simulink model "wind_resource_standalone"  (R2023b)
settings: Solver=ode23t  StartTime=0.0  StopTime=1.0  MaxStep=1e-5  RelTol=1e-3
InitFcn:
  | root=fileparts(fileparts(fileparts(get_param(bdroot,'FileName')))); addpath(root); setup_v2_paths; define_resource_buses(true); define_v2_parameters(true); define_wind_test_fixture(true);
undefined symbols (not defined in the file): DiscIntNeverNeededParam, ee, GridTransformer, SM, Ts, V2
libraries: ee_lib x18, nesl_utility x17, fl_lib x5, eeSmAC1C x1
settings Model: Creator=fakebob2004  LastModifiedBy=fakebob2004
settings ModelReferenceCC: UpdateModelReferenceTargets=IfOutOfDate
settings RTWCC: GPUComputeCapability=5.0
settings ConfigComp: CovBoundaryAbsTol=1.0e-5
settings SimscapeCC: SimscapeNominalValues="[{\"value\":\"1\",\"unit\":\"A\"},{\"value\":\"1\",\"unit\":\"bar\"},{\"value\":\"1\",\"unit\":\"cm^2\"},{\"value\":\"1\",\"unit\":\"cm^3/s\"},{\"value\":\"1\",\"unit\":\"kJ/kg\"},{\"value\":\"1\",\"unit\":\"kW\"},{\"value\":\"1\",\"unit\":\"l\"},{\"value\":\"1\",\"unit\":\"N\"},{\"value\":\"1\",\"unit\":\"N*m\"},{\"value\":\"1\",\"unit\":\"V\"},{\"value\":\"0.001\",\"unit\":\"Wb\"}]"  SimscapeLogType=all  SimscapeLogDataHistory=10000

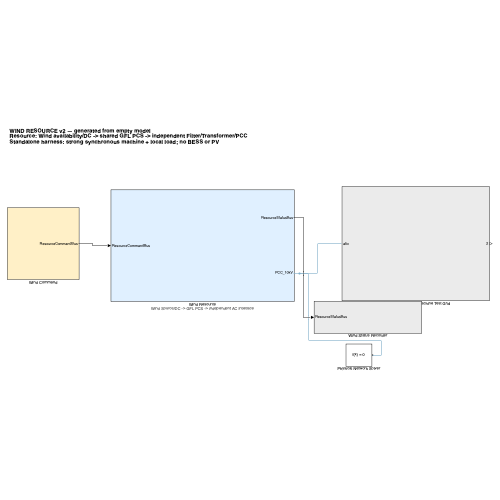
[thumbnail: Simulink's stored preview of the top-level diagram]
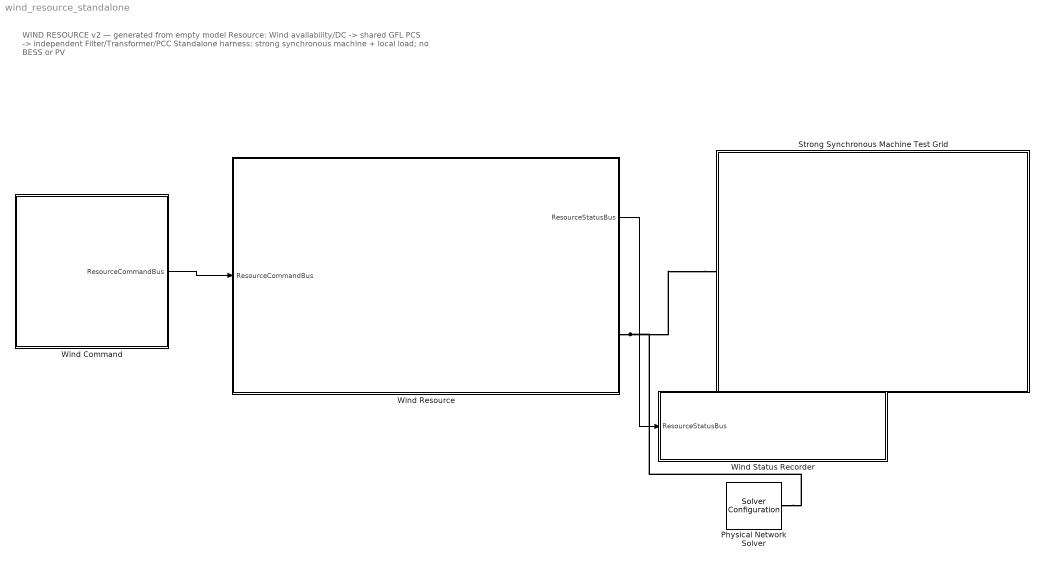
== system wind_resource_standalone ==
  note: WIND RESOURCE v2 — generated from empty model
      | Resource: Wind availability/DC -> shared GFL PCS -> independent Filter/Transformer/PCC
      | Standalone harness: strong synchronous machine + local load; no BESS or PV
  Physical Network Solver : nesl_utility/Solver Configuration  PhysicalDomain=network_engine_domain  SubClassName=solver  LeftPortType=input  RightPortType=generic  Tones=[]  Harmonics=[]  SimulateNoise=off  Profile=off  UseLocalSampling=off  EnableSwitchedLinearOptims=on  FrequencyDomain=off  UseCCode=off  RelTol=0.001  AbsTol=0.001  MinStep=1e-09  ToWorkspace=off  RevertToSquareIcSolve=off  NumHomotopyIterations=100  PhasorMode=off  PhasorModeNumHarmonics=1  ConsistencySolver=NEWTON_XTOL_AFTER_FTOL  CanonicalOrdering=CANONICAL  OptimizeIntermediates=OPTIMIZED  IndexReductionMethod=DerivativeReplacement  DoDC=off  ResidualTolerance=1e-09  ConsistencyTolSource=GLOBAL  ConsistencyAbsTol=0.001  ConsistencyRelTol=0.001  ConsistencyTolFactor=0.001  UseLocalSolver=off  LocalSolverChoice=NE_BACKWARD_EULER_ADVANCER  ResolveIndetEquations=on  FunctionEvalNumThread=1  LocalSolverSampleTime=0.001  DoFixedCost=off  MaxNonlinIter=3  MaxModeIter=2  ComputeImpulses=off  ImpulseIterations=2  LinearAlgebra=auto  LinearAlgebraNumThread=0  EquationFormulation=NE_TIME_EF  DelaysMemoryBudget=1024  AutomaticFiltering=on  FilteringTimeConstant=0.001  PartitionStorageMethod=AS_NEEDED  PartitionMemoryBudget=1024  PartitionMethod=ROBUST  MultibodyUseLocalSolver=off  MultibodyLocalSolverChoice=ODE1  MultibodyLocalSolverSampleTime=0.001
  Strong Synchronous Machine Test Grid : Subsystem  VariantControl=SynchronousMachine
  Wind Command : Subsystem
  Wind Resource : Subsystem
      settings: AttributesFormatString=Wind Source/DC -> GFL PCS -> independent AC Interface
  Wind Status Recorder : Subsystem
  wires:
  Wind Command/1(ResourceCommandBus) -> Wind Resource/1(ResourceCommandBus)
  Wind Resource/1(ResourceStatusBus) -> Wind Status Recorder/1(ResourceStatusBus)
  connections:
  Strong Synchronous Machine Test Grid/RConn1 -- Wind Resource/RConn1 -- Physical Network Solver/RConn1

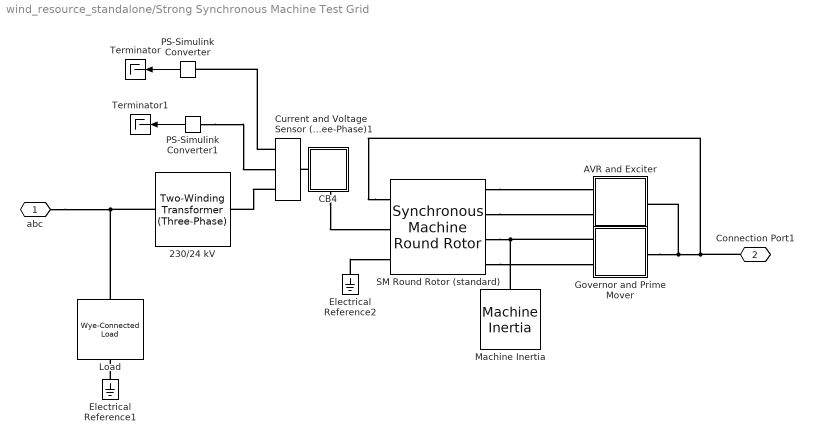
== system wind_resource_standalone/Strong Synchronous Machine Test Grid ==
  " Load" : ee_lib/Passive/RLC Assemblies/Wye-Connected Load  port_option=ee.enum.threePhasePort.composite  parameterization=ee.enum.rlc.parameterization.ratedpower  component_structure=ee.enum.rlc.structure.R  component_structure_PQ=ee.enum.rlc.structure.ParallelRL  R=1 Ohm  L=1e-3 H  C=1e-6 F  VRated=Grid.voltage V  FRated=Grid.frequency Hz  P=SM.P_load W  Qpos=SM.Q_load A*V  Qneg=-1e2 A*V  R_parasitic=0 Ohm  G_parasitic=0 1/Ohm  R_parasitic_PQ=0 Ohm  G_parasitic_PQ=0 1/Ohm  Vmag0=4.16e3 V  Vang0=0 deg  Freq0=60 Hz  IL_specify=off  IL_priority=High  IL=[0, 0, 0] A  IL_nominal_specify=off  IL_nominal_value=1  IL_nominal_unit=A  VC_specify=off  VC_priority=High  VC=[0, 0, 0] V  VC_nominal_specify=off  VC_nominal_value=1  VC_nominal_unit=V
  230/24 kV : ee_lib/Passive/Transformers/Two-Winding Transformer (Three-Phase)  SRated=SM.MVA V*A  FRated=Grid.frequency Hz  Winding1Connection=ee.enum.windingconnection.delta1  VRated1=Grid.voltage V  Winding2Connection=ee.enum.windingconnection.delta11  VRated2=SM.Voltage V  CoreType=ee.enum.coretype.fivelimb  pu_Rw1=GridTransformer.winding_resistance/2  pu_Rw2=GridTransformer.winding_resistance/2  leakage_reactance_option=ee.enum.transformer_leakage.include  pu_Xl1=GridTransformer.winding_lekage_reactance/2  pu_Xl2=GridTransformer.winding_lekage_reactance/2  magnetizing_resistance_option=ee.enum.transformer_magnetizingResistance.exclude  pu_Rm=500  magnetizing_reactance_option=ee.enum.transformer_magnetizingReactance.include  saturation_option=ee.enum.transformer_saturation.exclude  pu_Xm=500  current_data=[0, .002, 1, 2]  magnetic_flux_data=[0, 1.2, 1.5, 1.51]  pu_X0=0.0586/2  i1_specify=off  i1_priority=None  i1=[ 0 0 0 ] A  i1_nominal_specify=off  i1_nominal_value=1  i1_nominal_unit=A  i2_specify=off  i2_priority=None  i2=[ 0 0 0 ] A  i2_nominal_specify=off  i2_nominal_value=1  i2_nominal_unit=A  phi_specify=off  phi_priority=None  phi=[ 0 0 0 ]  phi_nominal_specify=off  phi_nominal_value=1  phi_nominal_unit=1
  AVR and Exciter : Subsystem
  CB4 : Subsystem
      settings: PortSchema="{\"entries\":[{\"content\":{\"sides\":[{\"content\":{\"connectorIds\":[\"LConn1\"]},\"type\":\"ConnectorPlacement.EquallySpacedRectSide\",\"uuid\":\"24022911-97b6-486c-a625-f0780a134feb\"},{\"content\":{\"connectorIds\":[],\"side\":\"RIGHT\"},\"type\":\"ConnectorPlacement.EquallySpacedRectSide\",\"uuid\":\"1242aa8b-343b-4af2-8b96-dfa58505a53d\"},{\"content\":{\"connectorIds\":[],\"side\":\"TOP\"},\"type\":\"ConnectorPlacement.EquallySpacedRectSide\",\"uuid\":\"e73be2e9-5300-480f-914f-665ff518f6ad\"},{\"content\":{\"connectorIds\":[\"RConn1\"],\"side\":\"BOTTOM\"},\"type\":\"ConnectorPlacement.EquallySpacedRectSide\",\"uuid\":\"6525202c-c4e7-4c96-9421-427b801d0594\"}]},\"type\":\"ConnectorPlacement.EquallySpacedConnector\",\"uuid\":\"b455682c-e951-4ef6-bff8-cd3f50b315f1\"}],\"packageUris\":[\"http://schema.mathworks.com/mf0/Connector/R2020b\"],\"version\":\"1.0\"}"
      mask Display: image('$imagefile'); % Use "Edit Image" on toolstrip to change.
  Current and Voltage Sensor (Three-Phase)1 : ee_lib/Sensors & Transducers/Current and Voltage Sensor (Three-Phase)  port_option=ee.enum.threePhasePort.composite  vMeasurementType=ee.enum.vmeasurement.ll  outputUnit=ee.enum.unit.pu  SRated=100e6 A*V  VRated=4.16e3 V  I_specify=off  I_priority=None  I=[0, 0, 0] A  I_nominal_specify=off  I_nominal_value=1  I_nominal_unit=A  V_specify=off  V_priority=None  V=[0, 0, 0] V  V_nominal_specify=off  V_nominal_value=1  V_nominal_unit=V
  Electrical Reference1 : fl_lib/Electrical/Electrical Elements/Electrical Reference
  Electrical Reference2 : fl_lib/Electrical/Electrical Elements/Electrical Reference
  "Governor and Prime Mover " : Subsystem  mask(Governor and Prime Mover){pu_speed_reference=SM.speed_reference, droop_percentage=SM.droop_p, pu_load_reference_setpoint=SM.load_reference_set_point, T_G=SM.governor_time_constant, T_CH=SM.time_constsnt_steamchest, base_torque=SM.Base_Torque_SM, pu_torque0=SM.initial_torque}
      mask prompts: pu_speed_reference "Speed reference, (pu)"; droop_percentage "Percentage droop, (%)"; pu_load_reference_setpoint "Load reference setpoint, (pu)"; T_G "Time constant of governor, (s)"; T_CH "Time constant of main inlet volumes and steam chest, (s)"; base_torque "Base torque, (N*m)"; pu_torque0 "Initial torque, (pu)"
      mask help:
      | Implements a synchronous machine governor and prime mover. The prime mover is a non-reheat steam turbine.
      |
      | The input to the block is a per-unit synchronous machine measurement vector.
      |
      | R and C are mechanical rotational ports.
  Machine Inertia : ee_lib/Electromechanical/Mechanical/Machine Inertia  SRated=SM.MVA V*A  FRated=Grid.frequency Hz  nPolePairs=SM.polepairs  inertia_option=2  J=27548 kg*m^2  H=SM.inertia s  damper_option=2  D=39.0509 N*m/(rad/s)  pu_D=SM.damping  initialization_option=2  fMechanical0=60 Hz  fElectrical0=Grid.frequency Hz
  PS-Simulink Converter : nesl_utility/PS-Simulink Converter  PhysicalDomain=network_engine_domain  SubClassName=ps_output  LeftPortType=input  RightPortType=output  PseudoPeriodic=off  Frequencies=[]  VectorFormat=inherit  Unit=inherit  AffineConversion=off
  PS-Simulink Converter1 : nesl_utility/PS-Simulink Converter  PhysicalDomain=network_engine_domain  SubClassName=ps_output  LeftPortType=input  RightPortType=output  PseudoPeriodic=off  Frequencies=[]  VectorFormat=inherit  Unit=inherit  AffineConversion=off
  SM Round Rotor (standard) : ee_lib/Electromechanical/Synchronous/Synchronous Machine Round Rotor  port_option=ee.enum.threePhasePort.composite  SRated=SM.MVA V*A  VRated=SM.Voltage V  FRated=Grid.frequency Hz  nPolePairs=SM.polepairs  param_option=ee.enum.sm.parameterization.standard  fieldCircuitParameterization_option=2  baseEfd=92.95 V  baseIfd=SM.field_current A  zero_sequence=ee.enum.park.zerosequence.include  axes_param=ee.enum.rotorangle.qaxis  Ladu=1.66  Laqu=1.61  L0=0.15  Ll=0.15  Ra=SM.stator_resistance  Lfd=0.165  Rfd=0.0006  L1d=0.1713  R1d=0.0284  L1q=0.7252  R1q=0.00619  L2q=0.125  R2q=0.02368  Xl=SM.lekage_reactance  Xd=SM.xd  Xq=SM.xq  X0=0.15  Xdd=SM.xd_  Xqd=SM.xq_  Xddd=SM.xd_dash  Xqdd=SM.xq_dash  d_option=1  Td0d=SM.Tdo_ s  Tdd=1.3260 s  Td0dd=SM.Tdo_dash s  Tddd=0.0230 s  q_option=1  Tq0d=SM.Tqo_ s  Tqd=0.3693 s  Tq0dd=SM.Tqo_dash s  Tqdd=0.0269 s  saturation_option=0  saturation_ifd=[0.00, 0.48, 0.76, 1.38, 1.79]  saturation_Vag=[0.00, 0.80, 1.08, 1.31, 1.40]  initialization_option=2  source_type=ee.enum.sm.load_flow_source_type.Swing  Vmag0=SM.Voltage V  Vang0=0 deg  Pt0=SM.initial_Pe V*A  Qt0=SM.initial_Qe V*A  minimum_pu=0.95  phase_search_range=[-inf, inf] deg  gmin=1e-6 S  connection_option=int32(ee.enum.Connection.wye)  num_q_dampers=2  rotor_offset=-pi / 2 rad  pu_psid_specify=on  pu_psid_priority=High  pu_psid=0  pu_psid_nominal_specify=off  pu_psid_nominal_value=1  pu_psid_nominal_unit=1  pu_psiq_specify=on  pu_psiq_priority=High  pu_psiq=0  pu_psiq_nominal_specify=off  pu_psiq_nominal_value=1  pu_psiq_nominal_unit=1  pu_psifd_specify=on  pu_psifd_priority=High  pu_psifd=0  pu_psifd_nominal_specify=off  pu_psifd_nominal_value=1  pu_psifd_nominal_unit=1  pu_psi1d_specify=on  pu_psi1d_priority=High  pu_psi1d=0  pu_psi1d_nominal_specify=off  pu_psi1d_nominal_value=1  pu_psi1d_nominal_unit=1  pu_psi1q_specify=on  pu_psi1q_priority=High  pu_psi1q=0  pu_psi1q_nominal_specify=off  pu_psi1q_nominal_value=1  pu_psi1q_nominal_unit=1  pu_psi2q_specify=on  pu_psi2q_priority=High  pu_psi2q=0  pu_psi2q_nominal_specify=off  pu_psi2q_nominal_value=1  pu_psi2q_nominal_unit=1  angular_position_diff_specify=on  angular_position_diff_priority=High  angular_position_diff=0 deg  angular_position_diff_nominal_specify=off  angular_position_diff_nominal_value=1  angular_position_diff_nominal_unit=deg  Tmeas=298.15 K  alpha=3.93e-3 1/K  stator_thermal_mass=100 J/K  rotor_thermal_mass=200 J/K  temperatureA_specify=off  temperatureA_priority=High  temperatureA=25 degC  temperatureA_nominal_specify=off  temperatureA_nominal_value=1  temperatureA_nominal_unit=degC  temperatureB_specify=off  temperatureB_priority=High  temperatureB=25 degC  temperatureB_nominal_specify=off  temperatureB_nominal_value=1  temperatureB_nominal_unit=degC  temperatureC_specify=off  temperatureC_priority=High  temperatureC=25 degC  temperatureC_nominal_specify=off  temperatureC_nominal_value=1  temperatureC_nominal_unit=degC  temperatureR_specify=off  temperatureR_priority=High  temperatureR=25 degC  temperatureR_nominal_specify=off  temperatureR_nominal_value=1  temperatureR_nominal_unit=degC
  Terminator : Terminator
  Terminator1 : Terminator
  abc : PMIOPort  Side=Right
  Connection Port1 : PMIOPort  Port=2  Side=Left
  wires:
  PS-Simulink Converter1/1 -> Terminator1/1
  PS-Simulink Converter/1 -> Terminator/1
  connections:
  Electrical Reference2/LConn1 -- SM Round Rotor (standard)/RConn3
  CB4/RConn1 -- SM Round Rotor (standard)/RConn2
  PS-Simulink Converter1/LConn1 -- Current and Voltage Sensor (Three-Phase)1/RConn2
  Current and Voltage Sensor (Three-Phase)1/RConn3 -- 230/24 kV/RConn1
  SM Round Rotor (standard)/LConn2 -- AVR and Exciter/RConn2
  Electrical Reference1/LConn1 -- " Load"/RConn1
  CB4/LConn1 -- Current and Voltage Sensor (Three-Phase)1/LConn1
  SM Round Rotor (standard)/LConn1 -- AVR and Exciter/RConn1
  Current and Voltage Sensor (Three-Phase)1/RConn1 -- PS-Simulink Converter/LConn1
  SM Round Rotor (standard)/LConn4 -- "Governor and Prime Mover "/RConn2
  "Governor and Prime Mover "/RConn1 -- Machine Inertia/LConn1 -- SM Round Rotor (standard)/LConn3
  SM Round Rotor (standard)/RConn1 -- Connection Port1/RConn1 -- AVR and Exciter/LConn1 -- "Governor and Prime Mover "/LConn1
  230/24 kV/LConn1 -- abc/RConn1 -- " Load"/LConn1

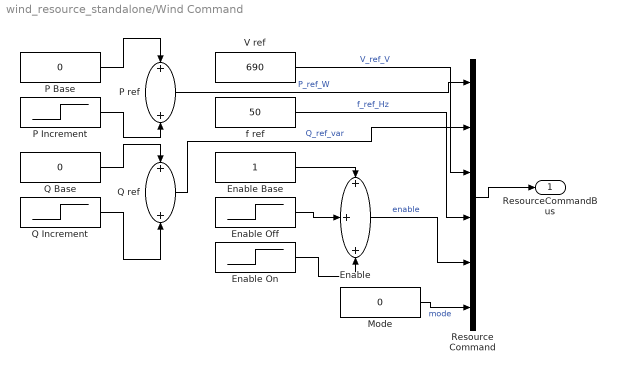
== system wind_resource_standalone/Wind Command ==
  Enable : Sum  Inputs=+++
  Enable Base : Constant
  Enable Off : Step  Time=10  After=-1  SampleTime=0
  Enable On : Step  Time=11  SampleTime=0
  Mode : Constant  Value=0
  P Base : Constant  Value=0
  P Increment : Step  Time=.30  After=2e6  SampleTime=0
  P ref : Sum
  Q Base : Constant  Value=0
  Q Increment : Step  Time=.30  After=0  SampleTime=0
  Q ref : Sum
  Resource Command : BusCreator  Inputs=6  OutDataTypeStr=Bus: ResourceCommandBus
  V ref : Constant  Value=690
  f ref : Constant  Value=50
  ResourceCommandBus : Outport  OutDataTypeStr=Bus: ResourceCommandBus
  wires:
  P Base/1 -> P ref/1
  P Increment/1 -> P ref/2
  Q Base/1 -> Q ref/1
  Q Increment/1 -> Q ref/2
  Enable Base/1 -> Enable/1
  Enable Off/1 -> Enable/2
  Enable On/1 -> Enable/3
  P ref/1 -> Resource Command/1  "P_ref_W"
  Q ref/1 -> Resource Command/2  "Q_ref_var"
  V ref/1 -> Resource Command/3  "V_ref_V"
  f ref/1 -> Resource Command/4  "f_ref_Hz"
  Enable/1 -> Resource Command/5  "enable"
  Mode/1 -> Resource Command/6  "mode"
  Resource Command/1 -> ResourceCommandBus/1

== system wind_resource_standalone/Wind Resource ==
  ResourceCommandBus : Inport  OutDataTypeStr=Bus: ResourceCommandBus
  01 Wind Source and DC Side : Subsystem
      settings: AttributesFormatString=replaceable by turbine + PMSG + MSC + physical DC link
  02 PCS : Subsystem
      settings: AttributesFormatString=local PLL | P/Q-to-dq | circle limit | average PCS
  03 AC Interface : Subsystem
      settings: AttributesFormatString=independent filter + 0.69/10 kV transformer + PCC sensing
  Status Interface : Subsystem
      settings: AttributesFormatString=typed local buses -> ResourceStatusBus
  PCC_10kV : PMIOPort  Side=Right  ConnectionType=Connection: foundation.electrical.three_phase
  ResourceStatusBus : Outport  OutDataTypeStr=Bus: ResourceStatusBus
  wires:
  ResourceCommandBus/1 -> 01 Wind Source and DC Side/1(ResourceCommandBus)
  01 Wind Source and DC Side/1(PCSCommandBus) -> 02 PCS/1(CommandBus)
  03 AC Interface/1(PCCMeasurementBus) -> 02 PCS/2(PCCMeasurementBus), Status Interface/3(PCC)
  01 Wind Source and DC Side/2(SourceStatusBus) -> Status Interface/1(Source)
  02 PCS/1(PCSStatusBus) -> Status Interface/2(PCS)
  Status Interface/1(ResourceStatusBus) -> ResourceStatusBus/1
  connections:
  02 PCS/RConn1 -- 03 AC Interface/LConn1
  03 AC Interface/RConn1 -- PCC_10kV/RConn1

== system wind_resource_standalone/Wind Status Recorder ==
  ResourceStatusBus : Inport  OutDataTypeStr=Bus: ResourceStatusBus
  Regression Vector : Mux  Inputs=12
  Status Selector : BusSelector  OutputSignals=P_W,Q_var,Vpcc_V,frequency_Hz,available_power_W,power_headroom_W,current_limit_factor,energy_state_pu,Vdc_V,control_mode,healthy
  Time : Clock
  Wind v2 Result : ToWorkspace  VariableName=wind_v2_result  SampleTime=-1
  wires:
  Time/1 -> Regression Vector/1
  Status Selector/1 -> Regression Vector/2  "<P_W>"
  Status Selector/2 -> Regression Vector/3  "<Q_var>"
  Status Selector/3 -> Regression Vector/4  "<Vpcc_V>"
  Status Selector/4 -> Regression Vector/5  "<frequency_Hz>"
  Status Selector/5 -> Regression Vector/6  "<available_power_W>"
  Status Selector/6 -> Regression Vector/7  "<power_headroom_W>"
  Status Selector/7 -> Regression Vector/8  "<current_limit_factor>"
  Status Selector/8 -> Regression Vector/9  "<energy_state_pu>"
  Status Selector/9 -> Regression Vector/10  "<Vdc_V>"
  Status Selector/10 -> Regression Vector/11  "<control_mode>"
  Status Selector/11 -> Regression Vector/12  "<healthy>"
  ResourceStatusBus/1 -> Status Selector/1
  Regression Vector/1 -> Wind v2 Result/1

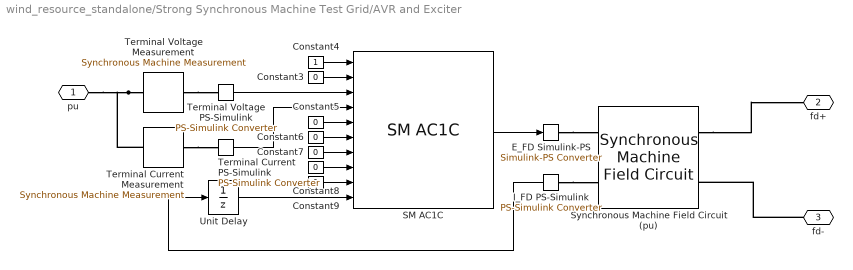
== system wind_resource_standalone/Strong Synchronous Machine Test Grid/AVR and Exciter ==
  Constant{3,5..9} (6 alike) : Constant  Value=0
  Constant4 : Constant
  "E_FD Simulink-PS " : nesl_utility/Simulink-PS Converter  PhysicalDomain=network_engine_domain  SubClassName=ps_input  LeftPortType=input  RightPortType=output  PseudoPeriodic=off  Frequencies=[]  NoiseDistribution=none  NoiseParameters=[]  Unit=1  AffineConversion=off  FilteringAndDerivatives=zero  SimscapeFilterOrder=1  InputFilterTimeConstant=.001  UdotUserProvided=0
  I_FD PS-Simulink : nesl_utility/PS-Simulink Converter  PhysicalDomain=network_engine_domain  SubClassName=ps_output  LeftPortType=input  RightPortType=output  PseudoPeriodic=off  Frequencies=[]  VectorFormat=1-D array  Unit=1  AffineConversion=off
  SM AC1C : eeSmAC1C/SM AC1C  E_FD0=1  Ts=-1  R_C=0  X_C=0  T_R=0  K_A=50  T_A=0.05  T_B=0  T_C=0  K_F=0.35  T_F=0.5  V_Amax=14.5  V_Amin=-14.5  E_FEmax=6.03  E_FEmin=-5.43  oelInputLocation=Unused  uelInputLocation=Unused  sclInputLocation=Unused  K_E=1  T_E=0.08  K_C=0.2  K_D=0.38  E_1=4.18  S_E_E1=0.1  E_2=3.14  S_E_E2=0.03  V_FEmax=99  V_Emin=0
  Synchronous Machine Field Circuit (pu) : ee_lib/Electromechanical/Synchronous/Synchronous Machine Field Circuit  unit_option=ee.enum.unit.pu  SRated=SM.MVA V*A  FRated=Grid.frequency Hz  fieldCircuitParameterization_option=2  baseEfd=92.95 V  baseIfd=1300 A  parameterization_option=2  Ladu=1.66  Rfd=0.0006  Xl=SM.lekage_reactance  Xd=SM.xd  Xdd=SM.xd_  Xddd=SM.xd_dash  d_option=ee.enum.circuit.open  Td0d=SM.Tdo_ s  Tdd=1.3260 s  Td0dd=SM.Tdo_dash s  Tddd=0.0230 s
  Terminal Current Measurement : ee_lib/Electromechanical/Synchronous/Synchronous Machine Measurement  output_idx=15
  Terminal Current PS-Simulink : nesl_utility/PS-Simulink Converter  PhysicalDomain=network_engine_domain  SubClassName=ps_output  LeftPortType=input  RightPortType=output  PseudoPeriodic=off  Frequencies=[]  VectorFormat=1-D array  Unit=1  AffineConversion=off
  Terminal Voltage Measurement : ee_lib/Electromechanical/Synchronous/Synchronous Machine Measurement  output_idx=14
  Terminal Voltage PS-Simulink : nesl_utility/PS-Simulink Converter  PhysicalDomain=network_engine_domain  SubClassName=ps_output  LeftPortType=input  RightPortType=output  PseudoPeriodic=off  Frequencies=[]  VectorFormat=1-D array  Unit=1  AffineConversion=off
  Unit Delay : UnitDelay  InitialCondition=1.32943  SampleTime=-1
  pu : PMIOPort  Side=Left
  fd+ : PMIOPort  Port=2  Side=Right
  fd- : PMIOPort  Port=3  Side=Right
  wires:
  I_FD PS-Simulink/1 -> Unit Delay/1
  Terminal Voltage PS-Simulink/1 -> SM AC1C/3
  Constant3/1 -> SM AC1C/2
  Constant4/1 -> SM AC1C/1
  Constant5/1 -> SM AC1C/5
  Constant6/1 -> SM AC1C/6
  Constant7/1 -> SM AC1C/7
  Constant8/1 -> SM AC1C/8
  Constant9/1 -> SM AC1C/9
  Unit Delay/1 -> SM AC1C/10
  SM AC1C/1 -> "E_FD Simulink-PS "/1
  Terminal Current PS-Simulink/1 -> SM AC1C/4
  connections:
  "E_FD Simulink-PS "/RConn1 -- Synchronous Machine Field Circuit (pu)/LConn1
  I_FD PS-Simulink/LConn1 -- Synchronous Machine Field Circuit (pu)/LConn2
  fd-/RConn1 -- Synchronous Machine Field Circuit (pu)/RConn2
  Synchronous Machine Field Circuit (pu)/RConn1 -- fd+/RConn1
  Terminal Voltage Measurement/LConn1 -- Terminal Current Measurement/LConn1 -- pu/RConn1
  Terminal Voltage Measurement/RConn1 -- Terminal Voltage PS-Simulink/LConn1
  Terminal Current Measurement/RConn1 -- Terminal Current PS-Simulink/LConn1

== system wind_resource_standalone/Strong Synchronous Machine Test Grid/CB4 ==
  Circuit Breaker Step off3 : ee_lib/Switches & Breakers/Circuit Breaker (Three-Phase)  port_option=ee.enum.threePhasePort.composite  control_port_option=ee.enum.controlport.ps  R_closed=0.001 Ohm  G_open=1e-4 1/Ohm  threshold=0.5 V  breaker_behavior=ee.enum.switches.breakerBehavior.zeroCrossingEnable  i_th=1e-8 A
  Simulink-PS Converter3 : nesl_utility/Simulink-PS Converter  PhysicalDomain=network_engine_domain  SubClassName=ps_input  LeftPortType=input  RightPortType=output  PseudoPeriodic=off  Frequencies=[]  NoiseDistribution=none  NoiseParameters=[]  Unit=1  AffineConversion=off  FilteringAndDerivatives=zero  SimscapeFilterOrder=1  InputFilterTimeConstant=0.001  UdotUserProvided=1
  Step off3 : Step  Time=0  After=0  SampleTime=Ts
  Conn2 : PMIOPort  Side=Left
  Conn1 : PMIOPort  Port=2  Side=Right
  wires:
  Step off3/1 -> Simulink-PS Converter3/1
  connections:
  Circuit Breaker Step off3/RConn1 -- Conn1/RConn1
  Circuit Breaker Step off3/LConn1 -- Simulink-PS Converter3/RConn1
  Circuit Breaker Step off3/LConn2 -- Conn2/RConn1

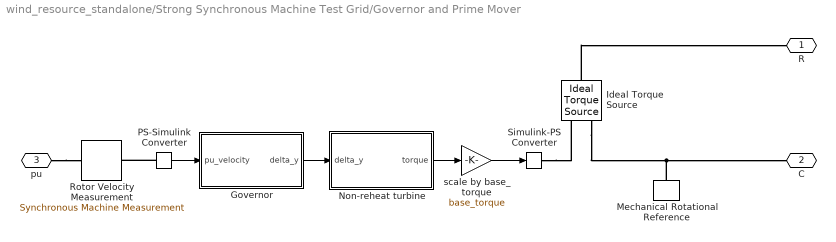
== system wind_resource_standalone/Strong Synchronous Machine Test Grid/Governor and Prime Mover  ==
  Governor : Subsystem
  Ideal Torque Source : fl_lib/Mechanical/Mechanical Sources/Ideal Torque Source
  Mechanical Rotational Reference : fl_lib/Mechanical/Rotational Elements/Mechanical Rotational Reference
  Non-reheat turbine : Subsystem
  PS-Simulink Converter : nesl_utility/PS-Simulink Converter  PhysicalDomain=network_engine_domain  SubClassName=ps_output  LeftPortType=input  RightPortType=output  PseudoPeriodic=off  Frequencies=[]  VectorFormat=1-D array  Unit=1  AffineConversion=off
  Rotor Velocity Measurement : ee_lib/Electromechanical/Synchronous/Synchronous Machine Measurement  output_idx=4
  Simulink-PS Converter : nesl_utility/Simulink-PS Converter  PhysicalDomain=network_engine_domain  SubClassName=ps_input  LeftPortType=input  RightPortType=output  PseudoPeriodic=off  Frequencies=[]  NoiseDistribution=none  NoiseParameters=[]  Unit=1  AffineConversion=off  FilteringAndDerivatives=zero  SimscapeFilterOrder=1  InputFilterTimeConstant=0.001  UdotUserProvided=1
  scale by base_torque : Gain  Gain=base_torque
  R : PMIOPort  Side=Right
  C : PMIOPort  Port=2  Side=Right
  pu : PMIOPort  Port=3  Side=Left
  wires:
  scale by base_torque/1 -> Simulink-PS Converter/1
  Non-reheat turbine/1(torque) -> scale by base_torque/1
  Governor/1(delta_y) -> Non-reheat turbine/1(delta_y)
  PS-Simulink Converter/1 -> Governor/1(pu_velocity)
  connections:
  Simulink-PS Converter/RConn1 -- Ideal Torque Source/RConn1
  PS-Simulink Converter/LConn1 -- Rotor Velocity Measurement/RConn1
  pu/RConn1 -- Rotor Velocity Measurement/LConn1
  Ideal Torque Source/LConn1 -- R/RConn1
  Mechanical Rotational Reference/LConn1 -- Ideal Torque Source/RConn2 -- C/RConn1

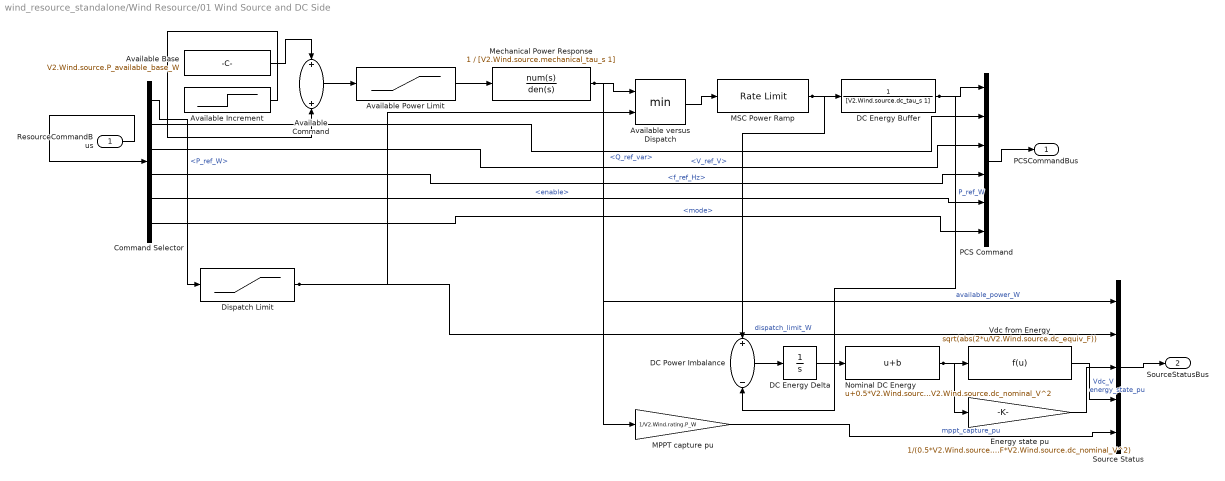
== system wind_resource_standalone/Wind Resource/01 Wind Source and DC Side ==
  ResourceCommandBus : Inport  OutDataTypeStr=Bus: ResourceCommandBus
  Available Base : Constant  Value=V2.Wind.source.P_available_base_W
  Available Command : Sum
  Available Increment : Step  Time=V2.Wind.source.P_available_step_time_s  After=V2.Wind.source.P_available_step_W  SampleTime=0
  Available Power Limit : Saturate  UpperLimit=V2.Wind.source.P_available_W  LowerLimit=0
  Available versus Dispatch : MinMax  Inputs=2
  Command Selector : BusSelector  OutputSignals=P_ref_W,Q_ref_var,V_ref_V,f_ref_Hz,enable,mode
  DC Energy Buffer : TransferFcn  Numerator=1  Denominator=[V2.Wind.source.dc_tau_s 1]
  DC Energy Delta : Integrator
  DC Power Imbalance : Sum  Inputs=+-
  Dispatch Limit : Saturate  UpperLimit=V2.Wind.rating.P_W  LowerLimit=0
  Energy state pu : Gain  Gain=1/(0.5*V2.Wind.source.dc_equiv_F*V2.Wind.source.dc_nominal_V^2)
  MPPT capture pu : Gain  Gain=1/V2.Wind.rating.P_W
  MSC Power Ramp : RateLimiter  RisingSlewLimit=V2.Wind.source.ramp_up_Wps  FallingSlewLimit=V2.Wind.source.ramp_down_Wps  SampleTimeMode=inherited
  Mechanical Power Response : TransferFcn  Numerator=1  Denominator=[V2.Wind.source.mechanical_tau_s 1]
  Nominal DC Energy : Bias  Bias=0.5*V2.Wind.source.dc_equiv_F*V2.Wind.source.dc_nominal_V^2  SaturateOnIntegerOverflow=off
  PCS Command : BusCreator  Inputs=6  OutDataTypeStr=Bus: ResourceCommandBus
  Source Status : BusCreator  Inputs=5  OutDataTypeStr=Bus: SourceStatusBus
  Vdc from Energy : Fcn  Expr=sqrt(abs(2*u/V2.Wind.source.dc_equiv_F))
  PCSCommandBus : Outport  OutDataTypeStr=Bus: ResourceCommandBus
  SourceStatusBus : Outport  Port=2  OutDataTypeStr=Bus: SourceStatusBus
  wires:
  ResourceCommandBus/1 -> Command Selector/1
  Available Base/1 -> Available Command/1
  Available Increment/1 -> Available Command/2
  Available Command/1 -> Available Power Limit/1
  Available Power Limit/1 -> Mechanical Power Response/1
  Command Selector/1 -> Dispatch Limit/1  "<P_ref_W>"
  Mechanical Power Response/1 -> Available versus Dispatch/1, MPPT capture pu/1, Source Status/1  "available_power_W"
  Dispatch Limit/1 -> Available versus Dispatch/2, Source Status/2  "dispatch_limit_W"
  Available versus Dispatch/1 -> MSC Power Ramp/1
  MSC Power Ramp/1 -> DC Energy Buffer/1, DC Power Imbalance/1
  DC Energy Buffer/1 -> PCS Command/1, DC Power Imbalance/2  "P_ref_W"
  Command Selector/2 -> PCS Command/2  "<Q_ref_var>"
  Command Selector/3 -> PCS Command/3  "<V_ref_V>"
  Command Selector/4 -> PCS Command/4  "<f_ref_Hz>"
  Command Selector/5 -> PCS Command/5  "<enable>"
  Command Selector/6 -> PCS Command/6  "<mode>"
  PCS Command/1 -> PCSCommandBus/1
  DC Power Imbalance/1 -> DC Energy Delta/1
  DC Energy Delta/1 -> Nominal DC Energy/1
  Nominal DC Energy/1 -> Vdc from Energy/1, Energy state pu/1
  Energy state pu/1 -> Source Status/3  "energy_state_pu"
  Vdc from Energy/1 -> Source Status/4  "Vdc_V"
  MPPT capture pu/1 -> Source Status/5  "mppt_capture_pu"
  Source Status/1 -> SourceStatusBus/1

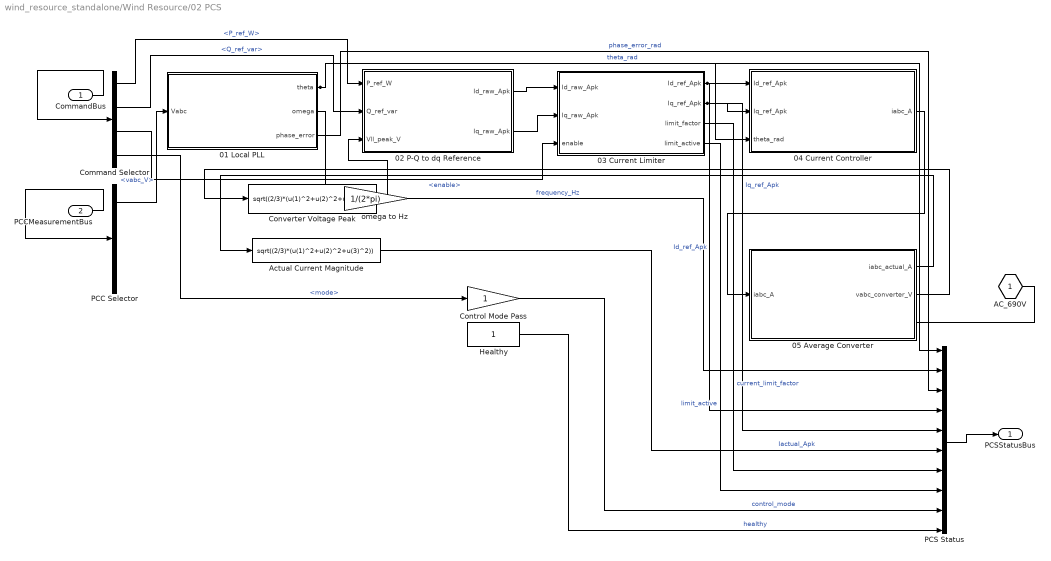
== system wind_resource_standalone/Wind Resource/02 PCS ==
  CommandBus : Inport  OutDataTypeStr=Bus: ResourceCommandBus
  PCCMeasurementBus : Inport  Port=2  OutDataTypeStr=Bus: PCCMeasurementBus
  01 Local PLL : Subsystem
      settings: AttributesFormatString=local PCC voltage only
  02 P-Q to dq Reference : Subsystem
  03 Current Limiter : Subsystem
  04 Current Controller : Subsystem
  05 Average Converter : Subsystem
  Actual Current Magnitude : Fcn  Expr=sqrt((2/3)*(u(1)^2+u(2)^2+u(3)^2))
  Command Selector : BusSelector  OutputSignals=P_ref_W,Q_ref_var,enable,mode
  Control Mode Pass : Gain
  Converter Voltage Peak : Fcn  Expr=sqrt((2/3)*(u(1)^2+u(2)^2+u(3)^2))
  Healthy : Constant
  PCC Selector : BusSelector  OutputSignals=vabc_V,iabc_A,Vll_rms_V
  PCS Status : BusCreator  Inputs=10  OutDataTypeStr=Bus: PCSStatusBus
  omega to Hz : Gain  Gain=1/(2*pi)
  AC_690V : PMIOPort  Side=Right  ConnectionType=Connection: foundation.electrical.three_phase
  PCSStatusBus : Outport  OutDataTypeStr=Bus: PCSStatusBus
  wires:
  CommandBus/1 -> Command Selector/1
  PCCMeasurementBus/1 -> PCC Selector/1
  PCC Selector/1 -> 01 Local PLL/1(Vabc)  "<vabc_V>"
  05 Average Converter/2(vabc_converter_V) -> Converter Voltage Peak/1
  Command Selector/1 -> 02 P-Q to dq Reference/1(P_ref_W)  "<P_ref_W>"
  Command Selector/2 -> 02 P-Q to dq Reference/2(Q_ref_var)  "<Q_ref_var>"
  Converter Voltage Peak/1 -> 02 P-Q to dq Reference/3(Vll_peak_V)
  02 P-Q to dq Reference/1(Id_raw_Apk) -> 03 Current Limiter/1(Id_raw_Apk)
  02 P-Q to dq Reference/2(Iq_raw_Apk) -> 03 Current Limiter/2(Iq_raw_Apk)
  Command Selector/3 -> 03 Current Limiter/3(enable)  "<enable>"
  03 Current Limiter/1(Id_ref_Apk) -> 04 Current Controller/1(Id_ref_Apk), PCS Status/4  "Id_ref_Apk"
  03 Current Limiter/2(Iq_ref_Apk) -> 04 Current Controller/2(Iq_ref_Apk), PCS Status/5  "Iq_ref_Apk"
  01 Local PLL/1(theta) -> 04 Current Controller/3(theta_rad), PCS Status/1  "theta_rad"
  04 Current Controller/1(iabc_A) -> 05 Average Converter/1(iabc_A)
  01 Local PLL/2(omega) -> omega to Hz/1
  05 Average Converter/1(iabc_actual_A) -> Actual Current Magnitude/1
  Command Selector/4 -> Control Mode Pass/1  "<mode>"
  omega to Hz/1 -> PCS Status/2  "frequency_Hz"
  01 Local PLL/3(phase_error) -> PCS Status/3  "phase_error_rad"
  Actual Current Magnitude/1 -> PCS Status/6  "Iactual_Apk"
  03 Current Limiter/3(limit_factor) -> PCS Status/7  "current_limit_factor"
  03 Current Limiter/4(limit_active) -> PCS Status/8  "limit_active"
  Control Mode Pass/1 -> PCS Status/9  "control_mode"
  Healthy/1 -> PCS Status/10  "healthy"
  PCS Status/1 -> PCSStatusBus/1
  connections:
  05 Average Converter/RConn1 -- AC_690V/RConn1

== system wind_resource_standalone/Wind Resource/03 AC Interface ==
  Damped Shunt C : ee_lib/Passive/RLC Assemblies/RLC (Three-Phase)  port_option=ee.enum.threePhasePort.composite  component_structure=ee.enum.rlc.structure.SeriesRC  R=V2.Wind.filter.Rd_ohm Ohm  L=1e-3 H  C=V2.Wind.filter.C_F F  R_parasitic=0 Ohm  G_parasitic=0 1/Ohm  IL_specify=off  IL_priority=High  IL=[0, 0, 0] A  IL_nominal_specify=off  IL_nominal_value=1  IL_nominal_unit=A  VC_specify=off  VC_priority=High  VC=[0, 0, 0] V  VC_nominal_specify=off  VC_nominal_value=1  VC_nominal_unit=V
  Equivalent Filter Series R : ee_lib/Passive/RLC Assemblies/RLC (Three-Phase)  port_option=ee.enum.threePhasePort.composite  component_structure=ee.enum.rlc.structure.R  R=V2.Wind.filter.R1_ohm+V2.Wind.filter.R2_ohm Ohm  L=1e-3 H  C=1e-6 F  R_parasitic=0 Ohm  G_parasitic=0 1/Ohm  IL_specify=off  IL_priority=High  IL=[0, 0, 0] A  IL_nominal_specify=off  IL_nominal_value=1  IL_nominal_unit=A  VC_specify=off  VC_priority=High  VC=[0, 0, 0] V  VC_nominal_specify=off  VC_nominal_value=1  VC_nominal_unit=V
  Filter Ground : ee_lib/Connectors & References/Grounded Neutral (Three-Phase)  port_option=ee.enum.threePhasePort.composite
  PCC Measurement : Subsystem
  Step-up Transformer : ee_lib/Passive/Transformers/Two-Winding Transformer (Three-Phase)  SRated=V2.Wind.transformer.S_VA A*V  FRated=V2.Wind.rating.f_Hz Hz  Winding1Connection=ee.enum.windingconnection.Yg  VRated1=V2.Wind.transformer.V1_V V  Winding2Connection=ee.enum.windingconnection.Yg  VRated2=V2.Wind.transformer.V2_V V  CoreType=ee.enum.coretype.threelimb  pu_Rw1=V2.Wind.transformer.R_pu/2  pu_Rw2=V2.Wind.transformer.R_pu/2  leakage_reactance_option=ee.enum.transformer_leakage.exclude  pu_Xl1=0.05  pu_Xl2=0.05  magnetizing_resistance_option=ee.enum.transformer_magnetizingResistance.exclude  pu_Rm=500  magnetizing_reactance_option=ee.enum.transformer_magnetizingReactance.exclude  saturation_option=ee.enum.transformer_saturation.exclude  pu_Xm=500  current_data=[0, .002, 1, 2]  magnetic_flux_data=[0, 1.2, 1.5, 1.51]  pu_X0=0.5  i1_specify=off  i1_priority=None  i1=[0, 0, 0] A  i1_nominal_specify=off  i1_nominal_value=1  i1_nominal_unit=A  i2_specify=off  i2_priority=None  i2=[0, 0, 0] A  i2_nominal_specify=off  i2_nominal_value=1  i2_nominal_unit=A  phi_specify=off  phi_priority=None  phi=[0, 0, 0]  phi_nominal_specify=off  phi_nominal_value=1  phi_nominal_unit=1
  PCS AC Terminal : PMIOPort  Side=Left  ConnectionType=Connection: foundation.electrical.three_phase
  PCC_10kV : PMIOPort  Port=2  Side=Right  ConnectionType=Connection: foundation.electrical.three_phase
  PCCMeasurementBus : Outport  OutDataTypeStr=Bus: PCCMeasurementBus
  wires:
  PCC Measurement/1(PCCMeasurementBus) -> PCCMeasurementBus/1
  connections:
  Equivalent Filter Series R/LConn1 -- PCS AC Terminal/RConn1 -- Damped Shunt C/LConn1
  Damped Shunt C/RConn1 -- Filter Ground/LConn1
  Equivalent Filter Series R/RConn1 -- Step-up Transformer/LConn1
  Step-up Transformer/RConn1 -- PCC Measurement/LConn1
  PCC Measurement/RConn1 -- PCC_10kV/RConn1

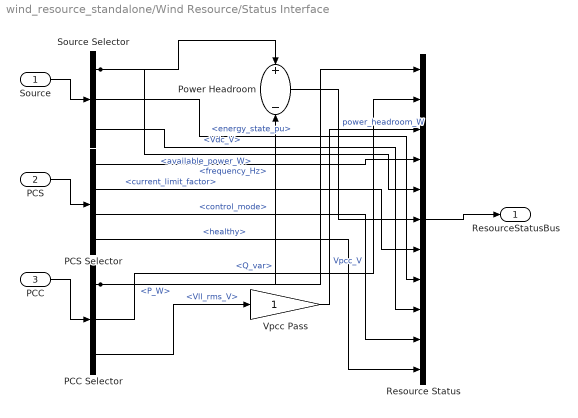
== system wind_resource_standalone/Wind Resource/Status Interface ==
  Source : Inport  OutDataTypeStr=Bus: SourceStatusBus
  PCS : Inport  Port=2  OutDataTypeStr=Bus: PCSStatusBus
  PCC : Inport  Port=3  OutDataTypeStr=Bus: PCCMeasurementBus
  PCC Selector : BusSelector  OutputSignals=P_W,Q_var,Vll_rms_V
  PCS Selector : BusSelector  OutputSignals=frequency_Hz,current_limit_factor,control_mode,healthy
  Power Headroom : Sum  Inputs=+-
  Resource Status : BusCreator  Inputs=11  OutDataTypeStr=Bus: ResourceStatusBus
  Source Selector : BusSelector  OutputSignals=available_power_W,energy_state_pu,Vdc_V
  Vpcc Pass : Gain
  ResourceStatusBus : Outport  OutDataTypeStr=Bus: ResourceStatusBus
  wires:
  PCC Selector/3 -> Vpcc Pass/1  "<Vll_rms_V>"
  Source/1 -> Source Selector/1
  PCS/1 -> PCS Selector/1
  PCC/1 -> PCC Selector/1
  Source Selector/1 -> Power Headroom/1, Resource Status/5  "<available_power_W>"
  PCC Selector/1 -> Power Headroom/2, Resource Status/1  "<P_W>"
  PCC Selector/2 -> Resource Status/2  "<Q_var>"
  Vpcc Pass/1 -> Resource Status/3  "Vpcc_V"
  PCS Selector/1 -> Resource Status/4  "<frequency_Hz>"
  Power Headroom/1 -> Resource Status/6  "power_headroom_W"
  PCS Selector/2 -> Resource Status/7  "<current_limit_factor>"
  Source Selector/2 -> Resource Status/8  "<energy_state_pu>"
  Source Selector/3 -> Resource Status/9  "<Vdc_V>"
  PCS Selector/3 -> Resource Status/10  "<control_mode>"
  PCS Selector/4 -> Resource Status/11  "<healthy>"
  Resource Status/1 -> ResourceStatusBus/1

== system wind_resource_standalone/Strong Synchronous Machine Test Grid/Governor and Prime Mover /Governor ==
  pu_velocity : Inport
  1/T_G : Gain  Gain=1/T_G
  1/droop : Gain  Gain=1/(droop_percentage/100)
  Delta load setpoint : Sum  Inputs=+-|
  Delta speed : Sum  Inputs=-+|
  Discrete-Time Integrator : DiscreteIntegrator  InitialCondition=pu_torque0  SampleTime=Ts  ICPrevOutput=DiscIntNeverNeededParam  ICPrevScaledInput=DiscIntNeverNeededParam
  Load_setpoint : Constant  Value=pu_load_reference_setpoint  SampleTime=Ts
  Speed_ref : Constant  Value=pu_speed_reference  SampleTime=Ts
  Subtract : Sum  Inputs=|+-
  delta_y : Outport  VectorParamsAs1DForOutWhenUnconnected=off
  wires:
  Discrete-Time Integrator/1 -> Subtract/2, delta_y/1
  1/T_G/1 -> Discrete-Time Integrator/1
  Subtract/1 -> 1/T_G/1
  Delta load setpoint/1 -> Subtract/1
  1/droop/1 -> Delta load setpoint/2
  pu_velocity/1 -> Delta speed/2
  Load_setpoint/1 -> Delta load setpoint/1
  Delta speed/1 -> 1/droop/1
  Speed_ref/1 -> Delta speed/1

== system wind_resource_standalone/Strong Synchronous Machine Test Grid/Governor and Prime Mover /Non-reheat turbine ==
  delta_y : Inport
  1/T_CH : Gain  Gain=1/T_CH
  Discrete-Time Integrator : DiscreteIntegrator  InitialCondition=pu_torque0  SampleTime=Ts  ICPrevOutput=DiscIntNeverNeededParam  ICPrevScaledInput=DiscIntNeverNeededParam
  Sum : Sum  Inputs=|+-
  torque : Outport  VectorParamsAs1DForOutWhenUnconnected=off
  wires:
  Discrete-Time Integrator/1 -> torque/1, Sum/2
  1/T_CH/1 -> Discrete-Time Integrator/1
  Sum/1 -> 1/T_CH/1
  delta_y/1 -> Sum/1

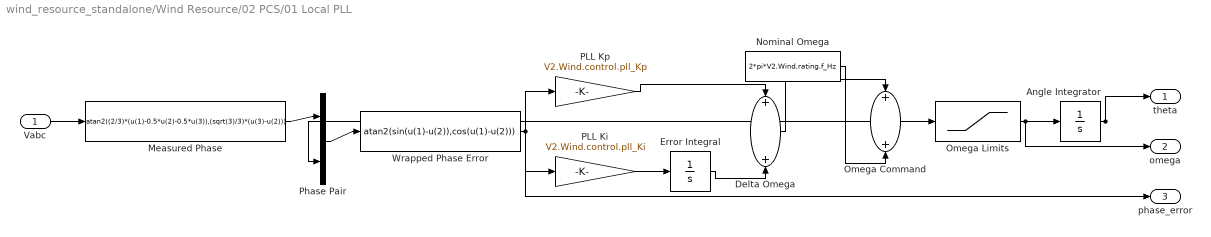
== system wind_resource_standalone/Wind Resource/02 PCS/01 Local PLL ==
  Vabc : Inport
  Angle Integrator : Integrator  InitialCondition=V2.Wind.control.pll_theta0_rad
  Delta Omega : Sum
  Error Integral : Integrator
  Measured Phase : Fcn  Expr=atan2((2/3)*(u(1)-0.5*u(2)-0.5*u(3)),(sqrt(3)/3)*(u(3)-u(2)))
  Nominal Omega : Constant  Value=2*pi*V2.Wind.rating.f_Hz
  Omega Command : Sum
  Omega Limits : Saturate  UpperLimit=2*pi*V2.Wind.control.pll_max_Hz  LowerLimit=2*pi*V2.Wind.control.pll_min_Hz
  PLL Ki : Gain  Gain=V2.Wind.control.pll_Ki
  PLL Kp : Gain  Gain=V2.Wind.control.pll_Kp
  Phase Pair : Mux  Inputs=2
  Wrapped Phase Error : Fcn  Expr=atan2(sin(u(1)-u(2)),cos(u(1)-u(2)))
  theta : Outport
  omega : Outport  Port=2
  phase_error : Outport  Port=3
  wires:
  Vabc/1 -> Measured Phase/1
  Measured Phase/1 -> Phase Pair/1
  Angle Integrator/1 -> Phase Pair/2, theta/1
  Phase Pair/1 -> Wrapped Phase Error/1
  Wrapped Phase Error/1 -> PLL Kp/1, PLL Ki/1, phase_error/1
  PLL Ki/1 -> Error Integral/1
  PLL Kp/1 -> Delta Omega/1
  Error Integral/1 -> Delta Omega/2
  Delta Omega/1 -> Omega Command/1
  Nominal Omega/1 -> Omega Command/2
  Omega Command/1 -> Omega Limits/1
  Omega Limits/1 -> Angle Integrator/1, omega/1

== system wind_resource_standalone/Wind Resource/02 PCS/02 P-Q to dq Reference ==
  P_ref_W : Inport
  Q_ref_var : Inport  Port=2
  Vll_peak_V : Inport  Port=3
  P and V : Mux  Inputs=2
  P to Id : Fcn  Expr=2*u(1)/(sqrt(3)*sqrt(u(2)^2+1))
  Q and V : Mux  Inputs=2
  Q to Iq : Fcn  Expr=-2*(u(1)-(2*pi*V2.Wind.rating.f_Hz*V2.Wind.filter.C_F/2)*u(2)^2)/(sqrt(3)*sqrt(u(2)^2+1))
  Id_raw_Apk : Outport
  Iq_raw_Apk : Outport  Port=2
  wires:
  P_ref_W/1 -> P and V/1
  Vll_peak_V/1 -> P and V/2, Q and V/2
  Q_ref_var/1 -> Q and V/1
  P and V/1 -> P to Id/1
  Q and V/1 -> Q to Iq/1
  P to Id/1 -> Id_raw_Apk/1
  Q to Iq/1 -> Iq_raw_Apk/1

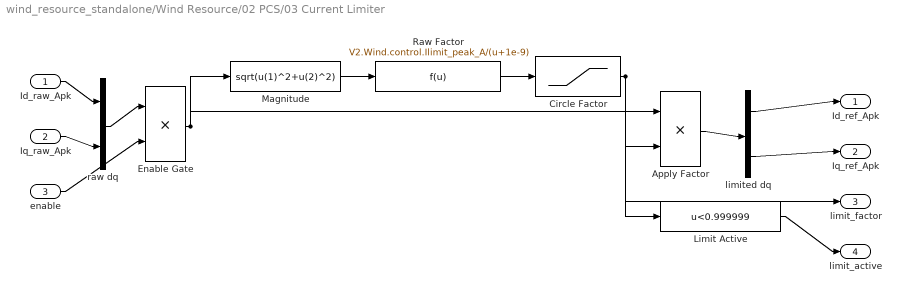
== system wind_resource_standalone/Wind Resource/02 PCS/03 Current Limiter ==
  Id_raw_Apk : Inport
  Iq_raw_Apk : Inport  Port=2
  enable : Inport  Port=3
  Apply Factor : Product
  Circle Factor : Saturate  UpperLimit=1  LowerLimit=0
  Enable Gate : Product
  Limit Active : Fcn  Expr=u<0.999999
  Magnitude : Fcn  Expr=sqrt(u(1)^2+u(2)^2)
  Raw Factor : Fcn  Expr=V2.Wind.control.Ilimit_peak_A/(u+1e-9)
  limited dq : Demux  Outputs=2
  raw dq : Mux  Inputs=2
  Id_ref_Apk : Outport
  Iq_ref_Apk : Outport  Port=2
  limit_factor : Outport  Port=3
  limit_active : Outport  Port=4
  wires:
  Id_raw_Apk/1 -> raw dq/1
  Iq_raw_Apk/1 -> raw dq/2
  raw dq/1 -> Enable Gate/1
  enable/1 -> Enable Gate/2
  Enable Gate/1 -> Magnitude/1, Apply Factor/1
  Magnitude/1 -> Raw Factor/1
  Raw Factor/1 -> Circle Factor/1
  Circle Factor/1 -> Apply Factor/2, limit_factor/1, Limit Active/1
  Apply Factor/1 -> limited dq/1
  limited dq/1 -> Id_ref_Apk/1
  limited dq/2 -> Iq_ref_Apk/1
  Limit Active/1 -> limit_active/1

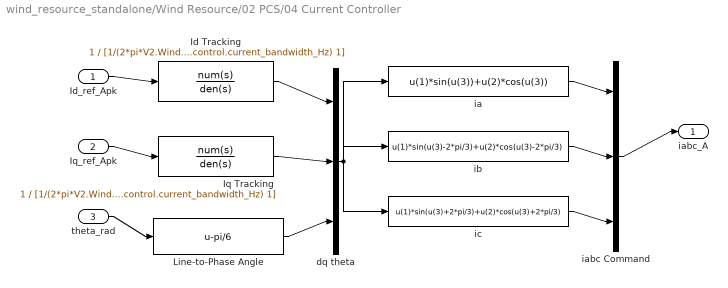
== system wind_resource_standalone/Wind Resource/02 PCS/04 Current Controller ==
  Id_ref_Apk : Inport
  Iq_ref_Apk : Inport  Port=2
  theta_rad : Inport  Port=3
  Id Tracking : TransferFcn  Numerator=1  Denominator=[1/(2*pi*V2.Wind.control.current_bandwidth_Hz) 1]
  Iq Tracking : TransferFcn  Numerator=1  Denominator=[1/(2*pi*V2.Wind.control.current_bandwidth_Hz) 1]
  Line-to-Phase Angle : Fcn  Expr=u-pi/6
  dq theta : Mux  Inputs=3
  ia : Fcn  Expr=u(1)*sin(u(3))+u(2)*cos(u(3))
  iabc Command : Mux  Inputs=3
  ib : Fcn  Expr=u(1)*sin(u(3)-2*pi/3)+u(2)*cos(u(3)-2*pi/3)
  ic : Fcn  Expr=u(1)*sin(u(3)+2*pi/3)+u(2)*cos(u(3)+2*pi/3)
  iabc_A : Outport
  wires:
  Id_ref_Apk/1 -> Id Tracking/1
  Iq_ref_Apk/1 -> Iq Tracking/1
  theta_rad/1 -> Line-to-Phase Angle/1
  Id Tracking/1 -> dq theta/1
  Iq Tracking/1 -> dq theta/2
  Line-to-Phase Angle/1 -> dq theta/3
  dq theta/1 -> ia/1, ib/1, ic/1
  ia/1 -> iabc Command/1
  ib/1 -> iabc Command/2
  ic/1 -> iabc Command/3
  iabc Command/1 -> iabc_A/1

== system wind_resource_standalone/Wind Resource/02 PCS/05 Average Converter ==
  iabc_A : Inport
  Average Current Injection : ee_lib/Sources/Controlled Current Source (Three-Phase)  port_option=ee.enum.threePhasePort.composite  input_option=ee.enum.inputType.instantaneous  FRated=V2.Wind.rating.f_Hz Hz  G_parasitic=1e-6 1/Ohm
  Converter Neutral : fl_lib/Electrical/Electrical Elements/Electrical Reference
  Converter-Side VI Sensor : ee_lib/Sensors & Transducers/Current and Voltage Sensor (Three-Phase)  port_option=ee.enum.threePhasePort.composite  vMeasurementType=ee.enum.vmeasurement.ll  outputUnit=ee.enum.unit.si  SRated=100e6 A*V  VRated=24e3 V  I_specify=off  I_priority=None  I=[0, 0, 0] A  I_nominal_specify=off  I_nominal_value=1  I_nominal_unit=A  V_specify=off  V_priority=None  V=[0, 0, 0] V  V_nominal_specify=off  V_nominal_value=1  V_nominal_unit=V
  Current Command to PS : nesl_utility/Simulink-PS Converter  PhysicalDomain=network_engine_domain  SubClassName=ps_input  LeftPortType=input  RightPortType=output  PseudoPeriodic=off  Frequencies=[]  NoiseDistribution=none  NoiseParameters=[]  Unit=A  AffineConversion=off  FilteringAndDerivatives=zero  SimscapeFilterOrder=1  InputFilterTimeConstant=0.001  UdotUserProvided=0
  iabc to Simulink : nesl_utility/PS-Simulink Converter  PhysicalDomain=network_engine_domain  SubClassName=ps_output  LeftPortType=input  RightPortType=output  PseudoPeriodic=off  Frequencies=[]  VectorFormat=inherit  Unit=A  AffineConversion=off
  vabc to Simulink : nesl_utility/PS-Simulink Converter  PhysicalDomain=network_engine_domain  SubClassName=ps_output  LeftPortType=input  RightPortType=output  PseudoPeriodic=off  Frequencies=[]  VectorFormat=inherit  Unit=V  AffineConversion=off
  AC_690V : PMIOPort  Side=Right  ConnectionType=Connection: foundation.electrical.three_phase
  iabc_actual_A : Outport
  vabc_converter_V : Outport  Port=2
  wires:
  iabc_A/1 -> Current Command to PS/1
  iabc to Simulink/1 -> iabc_actual_A/1
  vabc to Simulink/1 -> vabc_converter_V/1
  connections:
  Current Command to PS/RConn1 -- Average Current Injection/LConn1
  Average Current Injection/LConn2 -- Converter Neutral/LConn1
  Average Current Injection/RConn1 -- Converter-Side VI Sensor/LConn1
  Converter-Side VI Sensor/RConn3 -- AC_690V/RConn1
  Converter-Side VI Sensor/RConn2 -- iabc to Simulink/LConn1
  Converter-Side VI Sensor/RConn1 -- vabc to Simulink/LConn1

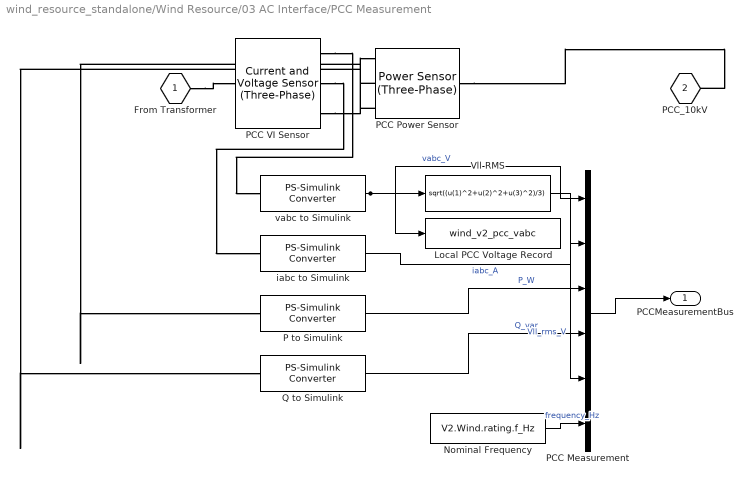
== system wind_resource_standalone/Wind Resource/03 AC Interface/PCC Measurement ==
  Local PCC Voltage Record : ToWorkspace  VariableName=wind_v2_pcc_vabc  SampleTime=-1
  Nominal Frequency : Constant  Value=V2.Wind.rating.f_Hz
  P to Simulink : nesl_utility/PS-Simulink Converter  PhysicalDomain=network_engine_domain  SubClassName=ps_output  LeftPortType=input  RightPortType=output  PseudoPeriodic=off  Frequencies=[]  VectorFormat=inherit  Unit=W  AffineConversion=off
  PCC Measurement : BusCreator  Inputs=6  OutDataTypeStr=Bus: PCCMeasurementBus
  PCC Power Sensor : ee_lib/Sensors & Transducers/Power Sensor (Three-Phase)  port_option=ee.enum.threePhasePort.composite  load_type=ee.enum.passive.type_balanced.balanced  f0=60 Hz
  PCC VI Sensor : ee_lib/Sensors & Transducers/Current and Voltage Sensor (Three-Phase)  port_option=ee.enum.threePhasePort.composite  vMeasurementType=ee.enum.vmeasurement.ll  outputUnit=ee.enum.unit.si  SRated=100e6 A*V  VRated=24e3 V  I_specify=off  I_priority=None  I=[0, 0, 0] A  I_nominal_specify=off  I_nominal_value=1  I_nominal_unit=A  V_specify=off  V_priority=None  V=[0, 0, 0] V  V_nominal_specify=off  V_nominal_value=1  V_nominal_unit=V
  Q to Simulink : nesl_utility/PS-Simulink Converter  PhysicalDomain=network_engine_domain  SubClassName=ps_output  LeftPortType=input  RightPortType=output  PseudoPeriodic=off  Frequencies=[]  VectorFormat=inherit  Unit=W  AffineConversion=off
  Vll RMS : Fcn  Expr=sqrt((u(1)^2+u(2)^2+u(3)^2)/3)
  iabc to Simulink : nesl_utility/PS-Simulink Converter  PhysicalDomain=network_engine_domain  SubClassName=ps_output  LeftPortType=input  RightPortType=output  PseudoPeriodic=off  Frequencies=[]  VectorFormat=inherit  Unit=A  AffineConversion=off
  vabc to Simulink : nesl_utility/PS-Simulink Converter  PhysicalDomain=network_engine_domain  SubClassName=ps_output  LeftPortType=input  RightPortType=output  PseudoPeriodic=off  Frequencies=[]  VectorFormat=inherit  Unit=V  AffineConversion=off
  From Transformer : PMIOPort  Side=Left  ConnectionType=Connection: foundation.electrical.three_phase
  PCC_10kV : PMIOPort  Port=2  Side=Right  ConnectionType=Connection: foundation.electrical.three_phase
  PCCMeasurementBus : Outport  OutDataTypeStr=Bus: PCCMeasurementBus
  wires:
  vabc to Simulink/1 -> Vll RMS/1, Local PCC Voltage Record/1, PCC Measurement/1  "vabc_V"
  iabc to Simulink/1 -> PCC Measurement/2  "iabc_A"
  P to Simulink/1 -> PCC Measurement/3  "P_W"
  Q to Simulink/1 -> PCC Measurement/4  "Q_var"
  Vll RMS/1 -> PCC Measurement/5  "Vll_rms_V"
  Nominal Frequency/1 -> PCC Measurement/6  "frequency_Hz"
  PCC Measurement/1 -> PCCMeasurementBus/1
  connections:
  From Transformer/RConn1 -- PCC VI Sensor/LConn1
  PCC VI Sensor/RConn3 -- PCC Power Sensor/LConn1
  PCC Power Sensor/RConn1 -- PCC_10kV/RConn1
  PCC VI Sensor/RConn1 -- vabc to Simulink/LConn1
  PCC VI Sensor/RConn2 -- iabc to Simulink/LConn1
  PCC Power Sensor/LConn2 -- P to Simulink/LConn1
  PCC Power Sensor/LConn3 -- Q to Simulink/LConn1
